simulink model "Model_31_03_1"  (R2024b)
settings: Solver=ode4  StartTime=0.0  StopTime=100  FixedStep=0.1  RelTol=1e-3
values from neighbouring files (symbols this model uses):
  alpha_t = 0    [Code_31_03.m]
  c = 2.29    [Code_31_03.m]
  delta_trim = x_trim(2) * 180/pi    [Code_31_03.m]
  delta_z_t = 0.378    [Code_31_03.m]
  diff_delta_e = -1    [Code_31_03.m]
  g = 9.81    [Code_31_03.m]
  I_yy = 84309    [Code_31_03.m]
  m = 7484.4    [Code_31_03.m]
  rho_h_trim = 1.225    [Code_31_03.m]
  S = 0    [Code_31_03.m]
  T_trim = x_trim(3)    [Code_31_03.m]
  V = sqrt((x(1))^2 + (x(2))^2)    [Code_31_03.m]
  x0_ver = [u; w; 0; theta_trim*pi/180; h_trim]    [Code_31_03.m]
settings Model: Creator=baron  LastModifiedBy=baron

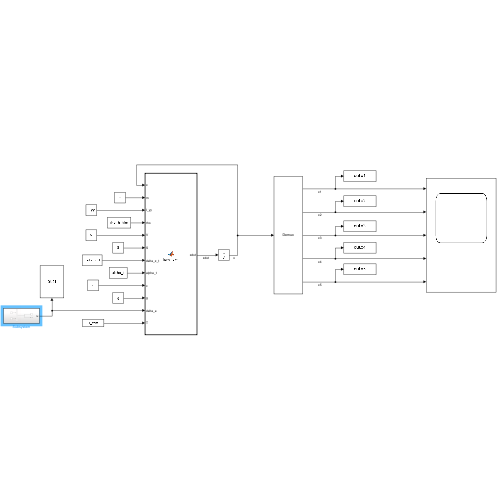
[thumbnail: Simulink's stored preview of the top-level diagram]
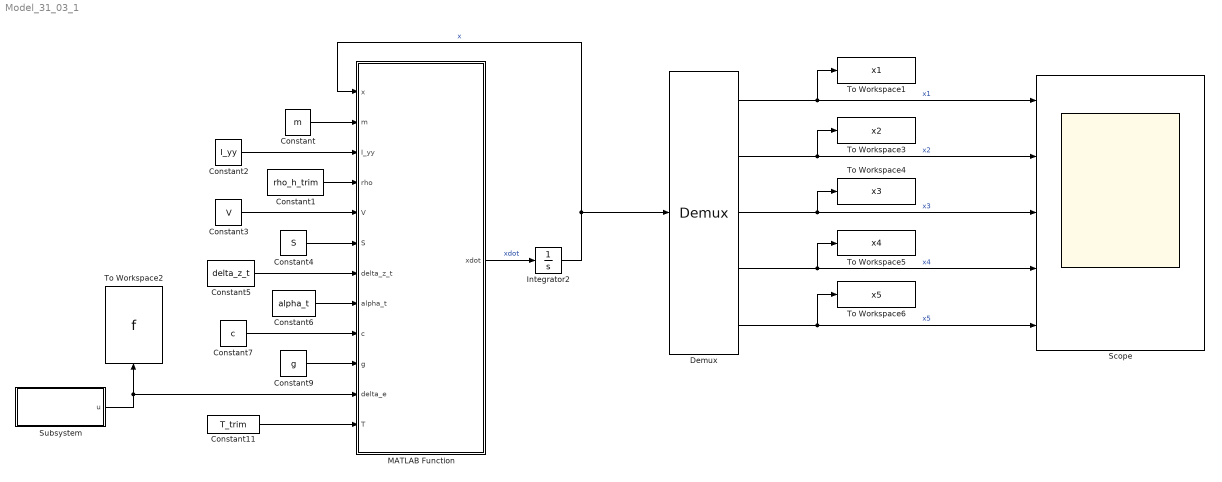
== system Model_31_03_1 ==
  Constant : Constant  Value=m
  Constant1 : Constant  Value=rho_h_trim
  Constant11 : Constant  Value=T_trim
  Constant2 : Constant  Value=I_yy
  Constant3 : Constant  Value=V
  Constant4 : Constant  Value=S
  Constant5 : Constant  Value=delta_z_t
  Constant6 : Constant  Value=alpha_t
  Constant7 : Constant  Value=c
  Constant9 : Constant  Value=g
  Demux : Demux  Outputs=5
      settings: DisplayOption=none
  Integrator2 : Integrator  InitialCondition=x0_ver
  MATLAB Function : MATLAB Function  TreatAsAtomicUnit=on
  Scope : Scope  NumInputPorts=5
  Subsystem : Subsystem
  To Workspace1 : ToWorkspace  VariableName=x1  SampleTime=-1
      settings: Save2DSignal=2-D array (concatenate along first dimension)
  To Workspace2 : ToWorkspace  VariableName=f  SampleTime=-1
      settings: Save2DSignal=2-D array (concatenate along first dimension)
  To Workspace3 : ToWorkspace  VariableName=x2  SampleTime=-1
      settings: Save2DSignal=2-D array (concatenate along first dimension)
  To Workspace4 : ToWorkspace  VariableName=x3  SampleTime=-1
      settings: Save2DSignal=2-D array (concatenate along first dimension)
  To Workspace5 : ToWorkspace  VariableName=x4  SampleTime=-1
      settings: Save2DSignal=2-D array (concatenate along first dimension)
  To Workspace6 : ToWorkspace  VariableName=x5  SampleTime=-1
      settings: Save2DSignal=2-D array (concatenate along first dimension)
  wires:
  Integrator2/1 -> MATLAB Function/1(x), Demux/1  "x"
  MATLAB Function/1(xdot) -> Integrator2/1  "xdot"
  Constant/1 -> MATLAB Function/2(m)
  Constant1/1 -> MATLAB Function/4(rho)
  Constant2/1 -> MATLAB Function/3(I_yy)
  Constant3/1 -> MATLAB Function/5(V)
  Constant4/1 -> MATLAB Function/6(S)
  Constant5/1 -> MATLAB Function/7(delta_z_t)
  Constant6/1 -> MATLAB Function/8(alpha_t)
  Constant7/1 -> MATLAB Function/9(c)
  Constant9/1 -> MATLAB Function/10(g)
  Constant11/1 -> MATLAB Function/12(T)
  Subsystem/1(u) -> To Workspace2/1, MATLAB Function/11(delta_e)
  Demux/3 -> Scope/3, To Workspace4/1  "x3"
  Demux/2 -> Scope/2, To Workspace3/1  "x2"
  Demux/1 -> To Workspace1/1, Scope/1  "x1"
  Demux/4 -> Scope/4, To Workspace5/1  "x4"
  Demux/5 -> Scope/5, To Workspace6/1  "x5"

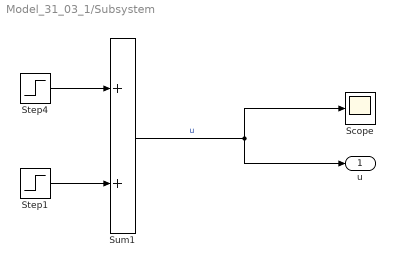
== system Model_31_03_1/Subsystem ==
  Scope : Scope
  Step1 : Step  Time=10  After=-diff_delta_e * pi / 180  SampleTime=0
  Step4 : Step  Time=5  Before=delta_trim * pi / 180  After=(diff_delta_e + delta_trim) * pi / 180  SampleTime=0
  Sum1 : Sum
  u : Outport
  wires:
  Sum1/1 -> u/1, Scope/1  "u"
  Step4/1 -> Sum1/1
  Step1/1 -> Sum1/2

== matlab function Model_31_03_1/MATLAB Function ==
  data: x input; m input; xdot output; I_yy input; rho input; V input; S input; delta_z_t input; alpha_t input; c input; g input; delta_e input; T input; coeff parameter
function xdot  = long_dyn(x, m, I_yy, rho, V, S, delta_z_t, alpha_t, c, g, delta_e, T, coeff)

    u = x(1); 
    w = x(2);
    q = x(3);
    theta = x(4);
    % h = x(5);     % variabile non utilizzata

    alpha = atan(x(2)/x(1)); 
    V = sqrt(x(1)^2 + x(2)^2);
    
    % coefficienti 
    CL = coeff.CL_0 + coeff.CL_alpha * alpha + coeff.CL_e * delta_e;
    CD = coeff.CD_0 + coeff.CD_alpha * alpha + coeff.CD_alpha2 * alpha^2;
    CM = coeff.CM_0 + coeff.CM_alpha * alpha + coeff.CM_e * delta_e + coeff.CM_q * c/V * q;


    % Forze
    D = 0.5 * rho * V^2 * S * CD; % Resistenza
    M = 0.5 * rho * V^2 * S * c * CM; % Momento rispetto al CG
    L = 0.5 * rho * V^2 * S * CL; % Portanza 
    S = 0; % Devianza

    % D S L sono validi eslcusivamente in asse wind, è quindi necessario
    % trasportarli, attraverso una matrice di rotazione, in asse body,
    % poiche le equazioni della dinamica longitudinale sono in tale sistema
    % di riferimento

    f_A = [-D; S; -L]; % Forze aerodinamiche

    % Matrice di passaggio asse body-wind
    C_bw = [cos(alpha) 0 -sin(alpha);
        0 1 0;
        sin(alpha) 0 cos(alpha)];

    % Forze aerodinamiche in asse body 
    X_A = [1 0 0] * (C_bw * f_A);
    X_T = T * cos(alpha_t);
    Z_A = [0 0 1] * (C_bw * f_A);
    Z_T = T * sin(alpha_t);
    M_A = M;
    M_T = delta_z_t * T;

    xdot = zeros(5,1);
    xdot(1) = -q * w -g * sin(theta) + 1/m * X_A + 1/m * X_T; 
    xdot(2) = q * u + g * cos(theta) + 1/m * Z_A + 1/m * Z_T;
    xdot(3) = 1/I_yy * (M_A + M_T);
    xdot(4) = q; 
    xdot(5) = u * sin(theta) - w * cos(theta); 

end
